simulink library "Multibody_Multiphysics_Lib"  (R2025a)
settings: Solver=ode45  StartTime=0.0  StopTime=10.0  RelTol=1e-3  EnableMultiTasking=on
undefined symbols (not defined in the file or in its folder): pst_rOut, rod_rOut
libraries: fl_lib x36, sm_lib x12, forcesPS_lib x9, $bdroot x1
Description:
  | Simscape Multibody Multiphysics Library v4.1
  | Copyright 2013-2025 The MathWorks, Inc.
settings Model: Creator=smiller  LastModifiedBy=smiller
settings SolverCC: AlgebraicLoopSolver=TrustRegion
settings DataIOCC: LimitDataPoints=on  SaveFormat=Array  SignalLoggingSaveFormat=ModelDataLogs  ReturnWorkspaceOutputs=off
settings OptimizationCC: ReuseModelBlockBuffer=off  ExpressionDepthLimit=2147483647.0  LifeSpan=inf
settings DebuggingCC: UnderspecifiedInitializationDetection=Classic  MergeDetectMultiDrivingBlocksExec=none  SolverPrmCheckMsg=warning  FcnCallInpInsideContextMsg=warning  UnconnectedInputMsg=warning  UnconnectedOutputMsg=warning  UnconnectedLineMsg=warning  AllowSymbolicDim=off  StateNameClashWarn=warning  PregeneratedLibrarySubsystemCodeDiagnostic=none  SFUnexpectedBacktrackingDiag=warning  SFNoUnconditionalDefaultTransitionDiag=warning  SFExecutionAtInitializationDiag=none  ArithmeticOperatorsInVariantConditions=warning
settings HardwareCC: ProdBitPerPointer=32.0  ProdBitPerSizeT=32.0  ProdBitPerPtrDiffT=32.0  ProdLargestAtomicFloat=None  ProdIntDivRoundTo=Undefined  ProdEndianess=Unspecified  ProdWordSize=32.0  ProdHWDeviceType=32-bit Generic
settings ModelReferenceCC: EnableRefExpFcnMdlSchedulingChecks=on  PropagateSignalLabelsOutOfModel=off
settings SFSimCC: SimUseLocalCustomCode=off  CustomCodeUndefinedFunction=UseInterfaceOnly
settings RTWCC: RTWUseLocalCustomCode=off  GPUComputeCapability=3.5  DLArmComputeVersion=19.05
settings CodeAppCC: StateflowObjectComments=on
settings GRTTargetCC: TargetLangStandard=C89/C90 (ANSI)
settings ConfigComp: CovMetricSettings=dw  CovSaveCumulativeToWorkspaceVar=on  CovSaveSingleToWorkspaceVar=on  CovExternalEMLEnable=off  CovSFcnEnable=off

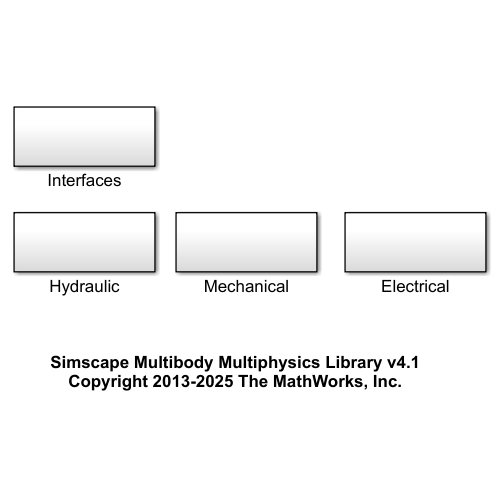
[thumbnail: Simulink's stored preview of the top-level diagram]
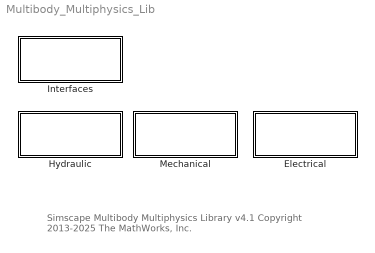
== system Multibody_Multiphysics_Lib ==
  note: Simscape Multibody Multiphysics Library v4.1
      | Copyright 2013-2025 The MathWorks, Inc.
  Electrical : Subsystem
  Hydraulic : Subsystem
  Interfaces : Subsystem
  Mechanical : Subsystem

== system Multibody_Multiphysics_Lib/Electrical ==
  DC Motor : Subsystem  Tag=PublishSubsystem

== system Multibody_Multiphysics_Lib/Hydraulic ==
  Hydraulic Actuator : Subsystem  mask(Double-Acting Hydraulic Cylinder, Kinematic Inputs){area_A=3e-4, area_B=1.57e-4, hs_stroke=0.1, hs_init_pos=0.01, dead_vol_A=1e-4, dead_vol_B=1e-4, popup_chamber_volume=Fixed, hs_stiffness=1e9, hs_damping=1500, friction_brkwy_frc=25, friction_brkwy_vel=0.1, friction_col_frc=20, friction_visc_coef=100}
      mask prompts: area_A "Piston Area A (m^2)"; area_B "Piston Area B (m^2)"; hs_stroke "Cylinder Stroke (m)"; hs_init_pos "Initial Position (m)"; dead_vol_A "Dead Volume Side A (m^3)"; dead_vol_B "Dead Volume Side B (m^3)"; popup_chamber_volume "Chamber Volume"; hs_stiffness "Hardstop Stiffness (N/m)"; hs_damping "Hardstop Damping (N/(m*s))"; friction_brkwy_frc "Breakaway Friction Force (N)"; friction_brkwy_vel "Breakaway Friction Velocity (m/s)"; friction_col_frc "Coulomb Friction Force (N)"; friction_visc_coef "Viscous Friction Coeff. (N/(m/s))"
      mask help:
      | Models a double-acting hydraulic cylinder with hardstops and compressibility.
      |
      | The position (m) and velocity (m/s) of the piston are inputs to this model.  This is to simplify the integration of this component with a Simscape Multibody joint.
      mask init:
      | temp_blk_h = gcb;
      | set_param([temp_blk_h '/Chamber A'],'dynamic_compressibility',num2str(popup_chamber_volume-1));
      | set_param([temp_blk_h '/Chamber B'],'dynamic_compressibility',num2str(popup_chamber_volume-1));
      | clear temp_blk_h
      mask TypeOptions popup_chamber_volume: Fixed | Varying
      mask DialogControl Container6 Prompt: Hydraulic
      mask DialogControl Container7 Prompt: Hardstop
      mask DialogControl Container8 Prompt: Friction
      mask Display:
      | color('white')
      | plot(-30,113.854429218918+10);
      | plot(326.445687096566+30,0);
      | color('black')
      | plot([127.790967235342;156.136468285695;156.136468285695;127.790967235342;127.790967235342], [113.618216710165;113.618216710165;56.927214609459;56.927214609459;113.618216710165])
      | plot([227.000220911577;227.000220911577;56.927214609459;56.927214609459;227.000220911577;227.000220911577], [99.4454661849886;113.618216710165;113.618216710165;56.927214609459;56.927214609459;71.0999651346356])
      | plot([156.136468285695;297.86397353746;297.86397353746;156.136468285695;156.136468285695], [99.4454661849886;99.4454661849886;71.0999651346356;71.0999651346356;99.4454661849886])
      | plot([56.927214609459;28.581713559106;56.927214609459], [113.618216710165;85.2727156598121;56.927214609459])
      | plot([28.581713559106;0.236212508752942], [85.2727156598121;85.2727156598121])
      | plot([297.86397353746;326.209474587813], [85.2727156598121;85.2727156598121])
      | plot([0.236212508752942;71.0999651346356;71.0999651346356], [28.581713559106;28.581713559106;56.927214609459])
      | plot([212.827470386401;212.827470386401;323.374924482778], [56.927214609459;28.581713559106;28.581713559106])
  Hydraulic Actuator PS FLib : Subsystem  Tag=PublishSubsystem  mask(Double-Acting Hydraulic Cylinder, PS Ports){area_A=pi*(pst_rOut/100)^2, area_B=pi*((pst_rOut/100)^2-(rod_rOut/100^2)), dead_vol_A=1e-4, dead_vol_B=1e-4, popup_chamber_volume=Fixed, p0_A=0, p0_B=0, friction_brkwy_frc=25, friction_brkwy_vel=0.1, friction_col_frc=20, friction_visc_coef=100}
      mask prompts: area_A "Piston Area A (m^2)"; area_B "Piston Area B (m^2)"; dead_vol_A "Dead Volume Side A (m^3)"; dead_vol_B "Dead Volume Side B (m^3)"; popup_chamber_volume "Chamber Volume"; p0_A "Initial Pressure A (Pa)"; p0_B "Initial Pressure B (Pa)"; friction_brkwy_frc "Breakaway Friction Force (N)"; friction_brkwy_vel "Breakaway Friction Velocity (m/s)"; friction_col_frc "Coulomb Friction Force (N)"; friction_visc_coef "Viscous Friction Coeff. (N/(m/s))"
      mask help:
      | Models a double-acting hydraulic cylinder with compressibility.
      |
      | The position (m) and velocity (m/s) of the piston are inputs to this model.  This is to simplify the integration of this component with a Simscape Multibody joint.
      mask init:
      | temp_blk_h = gcb;
      | set_param([temp_blk_h '/Chamber A'],'dynamic_compressibility',num2str(popup_chamber_volume-1));
      | set_param([temp_blk_h '/Chamber B'],'dynamic_compressibility',num2str(popup_chamber_volume-1));
      | clear temp_blk_h
      | 
      | % Parameter callback section
      mask TypeOptions popup_chamber_volume: Fixed | Varying
      mask DialogControl Container6 Prompt: Hydraulic
      mask DialogControl Container11 Prompt: Friction
      mask Display:
      | color('white')
      | plot(-30,113.854429218918+10);
      | plot(326.445687096566+30,0);
      | color('black')
      | plot([127.790967235342;156.136468285695;156.136468285695;127.790967235342;127.790967235342], [113.618216710165;113.618216710165;56.927214609459;56.927214609459;113.618216710165])
      | plot([227.000220911577;227.000220911577;56.927214609459;56.927214609459;227.000220911577;227.000220911577], [99.4454661849886;113.618216710165;113.618216710165;56.927214609459;56.927214609459;71.0999651346356])
      | plot([156.136468285695;297.86397353746;297.86397353746;156.136468285695;156.136468285695], [99.4454661849886;99.4454661849886;71.0999651346356;71.0999651346356;99.4454661849886])
      | plot([56.927214609459;28.581713559106;56.927214609459], [113.618216710165;85.2727156598121;56.927214609459])
      | plot([28.581713559106;0.236212508752942], [85.2727156598121;85.2727156598121])
      | plot([297.86397353746;326.209474587813], [85.2727156598121;85.2727156598121])
      | plot([0.236212508752942;71.0999651346356;71.0999651346356], [28.581713559106;28.581713559106;56.927214609459])
      | plot([212.827470386401;212.827470386401;323.374924482778], [56.927214609459;28.581713559106;28.581713559106])
  Hydraulic Actuator SA PS FLib : Subsystem  Tag=PublishSubsystem  mask(Double-Acting Hydraulic Cylinder, PS Ports){area_A=pi*(pst_rOut/100)^2, dead_vol_A=1e-4, popup_chamber_volume=Fixed, p0_A=0, friction_brkwy_frc=25, friction_brkwy_vel=0.1, friction_col_frc=20, friction_visc_coef=100}
      mask prompts: area_A "Piston Area A (m^2)"; dead_vol_A "Dead Volume Side A (m^3)"; popup_chamber_volume "Chamber Volume"; p0_A "Initial Pressure A (Pa)"; friction_brkwy_frc "Breakaway Friction Force (N)"; friction_brkwy_vel "Breakaway Friction Velocity (m/s)"; friction_col_frc "Coulomb Friction Force (N)"; friction_visc_coef "Viscous Friction Coeff. (N/(m/s))"
      mask help:
      | Models a double-acting hydraulic cylinder with hardstops and compressibility.
      |
      | The position (m) and velocity (m/s) of the piston are inputs to this model.  This is to simplify the integration of this component with a Simscape Multibody joint.
      mask init:
      | temp_blk_h = gcb;
      | set_param([temp_blk_h '/Chamber A'],'dynamic_compressibility',num2str(popup_chamber_volume-1));
      | clear temp_blk_h
      mask TypeOptions popup_chamber_volume: Fixed | Varying
      mask DialogControl Container6 Prompt: Hydraulic
      mask DialogControl Container11 Prompt: Friction
      mask Display:
      | color('white')
      | plot(-30,113.854429218918+10);
      | plot(326.445687096566+30,0);
      | color('black')
      | plot([127.790967235342;156.136468285695;156.136468285695;127.790967235342;127.790967235342], [113.618216710165;113.618216710165;56.927214609459;56.927214609459;113.618216710165])
      | plot([227.000220911577;227.000220911577;56.927214609459;56.927214609459;227.000220911577;227.000220911577], [99.4454661849886;113.618216710165;113.618216710165;56.927214609459;56.927214609459;71.0999651346356])
      | plot([156.136468285695;297.86397353746;297.86397353746;156.136468285695;156.136468285695], [99.4454661849886;99.4454661849886;71.0999651346356;71.0999651346356;99.4454661849886])
      | plot([56.927214609459;28.581713559106;56.927214609459], [113.618216710165;85.2727156598121;56.927214609459])
      | plot([28.581713559106;0.236212508752942], [85.2727156598121;85.2727156598121])
      | plot([297.86397353746;326.209474587813], [85.2727156598121;85.2727156598121])
      | plot([0.236212508752942;71.0999651346356;71.0999651346356], [28.581713559106;28.581713559106;56.927214609459])
      | plot([212.827470386401;212.827470386401;323.374924482778], [56.927214609459;28.581713559106;28.581713559106])

== system Multibody_Multiphysics_Lib/Interfaces ==
  Rotational Simscape Intf : Subsystem
  Rotational Simscape Multibody : Subsystem
  Translational Simscape Intf : Subsystem
  Translational Simscape Multibody : Subsystem

== system Multibody_Multiphysics_Lib/Mechanical ==
  Rotational Hard Stop Friction : Subsystem  Tag=PublishSubsystem  mask(Rotational Hard Stop and Friction, Multibody Ports){hs_upper_bnd=45*pi/180, hs_lower_bnd=-45*pi/180, hs_stiffness=1e6, hs_damping=1e2, friction_brkwy_trq=2.5, friction_brkwy_vel=0.1, friction_col_trq=2, friction_visc_coeff=0.001}
      mask prompts: hs_upper_bnd "Max Angular Position (rad)"; hs_lower_bnd "Min Angular Position (rad)"; hs_stiffness "Hardstop Stiffness (N*m/rad)"; hs_damping "Hardstop Damping (N*m/(rad/s))"; friction_brkwy_trq "Breakaway Friction Torque (N*m)"; friction_brkwy_vel "Breakaway Friction Velocity (rad/s)"; friction_col_trq "Coulomb Friction Torque (N*m)"; friction_visc_coeff "Viscous Friction Coeff. (N*m/(rad/s))"
      mask help:
      | Hardstops and friction for use with rotational degrees of freedom in Simscape Multibody.
      |
      | Connect the mechanical ports in parallel with a Simscape Multibody joint that has a rotational degree of freedom.
      |
      | 1. Connect B and F ports to joint B and F ports, respectively
      | 2. Orient joint frames so rotation range is (lower -- upper)
      mask DialogControl Container15 Prompt: Hardstop
      mask DialogControl Container16 Prompt: Friction
  Rotational Hard Stop Friction PS : Subsystem  Tag=PublishSubsystem  mask(Rotational Hard Stop and Friction, PS Ports){hs_upper_bnd=45*pi/180, hs_lower_bnd=-45*pi/180, hs_stiffness=1e6, hs_damping=1e2, friction_brkwy_trq=2.5, friction_brkwy_vel=0.1, friction_col_trq=2, friction_visc_coef=0.001}
      mask prompts: hs_upper_bnd "Max Angular Position (rad)"; hs_lower_bnd "Min Angular Position (rad)"; hs_stiffness "Hardstop Stiffness (N*m/rad)"; hs_damping "Hardstop Damping (N*m/(rad/s))"; friction_brkwy_trq "Breakaway Friction Torque (N*m)"; friction_brkwy_vel "Breakaway Friction Velocity (rad/s)"; friction_col_trq "Coulomb Friction Force (N*m)"; friction_visc_coef "Viscous Friction Coeff. (N*m/(rad/s))"
      mask help:
      | Hardstops and friction force for use with rotational degrees of freedom in Simscape Multibody.
      |
      | Connect the physical signal ports to measurements from a Simscape Multibody joint with a rotational degree of freedom.  Apply the calculated torque to the frames used in the joint, either via joint actuation or torque blocks.
      |
      | 1. Connect B and F ports to joint B and F ports, respectively
      | 2. Orient joint frames so extension range is (0 -- stroke)
      mask DialogControl Container15 Prompt: Hardstop
      mask DialogControl Container16 Prompt: Friction
  Translational Hard Stop Friction : Subsystem  Tag=PublishSubsystem  mask(Translational Hard Stop and Friction, Multibody Ports){stroke=0.7, stiffness=1e9, damping=1.5e8, friction_breakaway=0.2, friction_brkwy_vel=0.1, friction_coulomb=0.2, friction_viscous=1*0.01}
      mask prompts: stroke "Distance Between Stops (m)"; stiffness "Hardstop Stiffness (N/m)"; damping "Hardstop Damping (N/(m*s))"; friction_breakaway "Breakaway Friction Force (N)"; friction_brkwy_vel "Breakaway Friction Velocity (m/s)"; friction_coulomb "Coulomb Friction Force (N)"; friction_viscous "Viscous Friction Coeff. (N/(m/s))"
      mask help:
      | Hardstops and friction for use with translational degrees of freedom in Simscape Multibody.
      |
      | Connect the mechanical ports in parallel with a Simscape Multibody joint that has a translational degree of freedom.
      |
      | 1. Connect B and F ports to joint B and F ports, respectively
      | 2. Orient joint frames so extension range is (0 -- distance)
      mask DialogControl Container15 Prompt: Hardstop
      mask DialogControl Container16 Prompt: Friction
  Translational Hard Stop Friction PS : Subsystem  mask(Translational Hard Stop and Friction, PS Ports){hs_stroke=0.1, hs_stiffness=1e6, hs_damping=1500, friction_brkwy_frc=25, friction_brkwy_vel=0.1, friction_col_frc=20, friction_visc_coef=100}
      mask prompts: hs_stroke "Distance between stops (m)"; hs_stiffness "Hardstop Stiffness (N/m)"; hs_damping "Hardstop Damping (N/(m*s))"; friction_brkwy_frc "Breakaway Friction Force (N)"; friction_brkwy_vel "Breakaway Friction Velocity (m/s)"; friction_col_frc "Coulomb Friction Force (N)"; friction_visc_coef "Viscous Friction Coeff. (N/(m/s))"
      mask help:
      | Hardstops and friction force for use with translational degrees of freedom in Simscape Multibody.
      |
      | Connect the physical signal ports to measurements from a Simscape Multibody joint with a translational degree of freedom.  Apply the calculated force to the frames used in the joint, either via joint actuation or force blocks.
      |
      | 1. Connect B and F ports to joint B and F ports, respectively
      | 2. Orient joint frames so extension range is (0 -- distance)
      mask DialogControl Container15 Prompt: Hardstop
      mask DialogControl Container16 Prompt: Friction

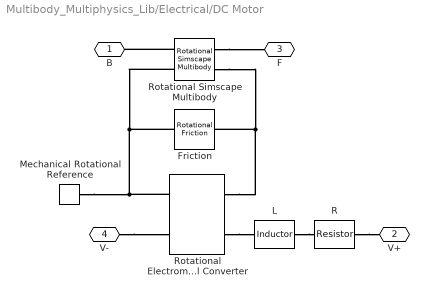
== system Multibody_Multiphysics_Lib/Electrical/DC Motor ==
  Friction : fl_lib/Mechanical/Rotational Elements/Rotational Friction  brkwy_trq=15e-3 N*m  brkwy_vel=0.057625 rad/s  Col_trq=5e-3 N*m  visc_coef=5e-3 N*m/(rad/s)  w_specify=off  w_priority=High  w=0 rad/s  w_nominal_specify=off  w_nominal_value=1  w_nominal_unit=rad/s  t_specify=off  t_priority=High  t=0 N*m  t_nominal_specify=off  t_nominal_value=1  t_nominal_unit=N*m
  L : fl_lib/Electrical/Electrical Elements/Inductor  l=12e-6 H  r=0 Ohm  g=1e-09 1/Ohm  i_specify=off  i_priority=High  i=0 A  i_nominal_specify=off  i_nominal_value=1  i_nominal_unit=A  v_specify=off  v_priority=High  v=0 V  v_nominal_specify=off  v_nominal_value=1  v_nominal_unit=V  i_L_specify=on  i_L_priority=High  i_L=0 A  i_L_nominal_specify=off  i_L_nominal_value=1  i_L_nominal_unit=A
  Mechanical Rotational Reference : fl_lib/Mechanical/Rotational Elements/Mechanical Rotational Reference
  R : fl_lib/Electrical/Electrical Elements/Resistor  Tag=Factory Generic  R=3.9 Ohm  i_specify=off  i_priority=High  i=0 A  i_nominal_specify=off  i_nominal_value=1  i_nominal_unit=A  v_specify=off  v_priority=High  v=0 V  v_nominal_specify=off  v_nominal_value=1  v_nominal_unit=V
  Rotational Electromechanical Converter : fl_lib/Electrical/Electrical Elements/Rotational Electromechanical Converter  K=0.072e-3*60/(2*pi)*20 V/(rad/s)  i_specify=off  i_priority=High  i=0 A  i_nominal_specify=off  i_nominal_value=1  i_nominal_unit=A  v_specify=off  v_priority=High  v=0 V  v_nominal_specify=off  v_nominal_value=1  v_nominal_unit=V  t_specify=off  t_priority=High  t=0 N*m  t_nominal_specify=off  t_nominal_value=1  t_nominal_unit=N*m  w_specify=off  w_priority=High  w=0 rad/s  w_nominal_specify=off  w_nominal_value=1  w_nominal_unit=rad/s
  Rotational Simscape Multibody : $bdroot/Interfaces/Rotational Simscape Multibody  Tag=PublishSubsystem  SystemSampleTime=-1  VariantActivationTime=update diagram  EmptyChoice=off  PassThrough=off  PassThroughVariantControl=(default)  EmptyChoiceVariantControl=(default)  AllowFlexibleInterface=on  Latency=0  AutoFrameSizeCalculation=off
  B : PMIOPort  Side=Left
  V+ : PMIOPort  Port=2  Side=Left
  F : PMIOPort  Port=3  Side=Right
  V- : PMIOPort  Port=4  Side=Right
  connections:
  Rotational Simscape Multibody/LConn1 -- B/RConn1
  Rotational Simscape Multibody/RConn1 -- F/RConn1
  Rotational Electromechanical Converter/LConn1 -- L/RConn1
  V-/RConn1 -- Rotational Electromechanical Converter/RConn1
  R/LConn1 -- V+/RConn1
  L/LConn1 -- R/RConn1
  Rotational Electromechanical Converter/LConn2 -- Rotational Simscape Multibody/RConn2 -- Friction/LConn1
  Mechanical Rotational Reference/LConn1 -- Rotational Electromechanical Converter/RConn2 -- Rotational Simscape Multibody/LConn2 -- Friction/RConn1

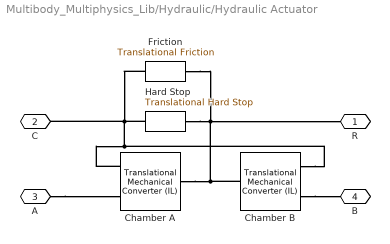
== system Multibody_Multiphysics_Lib/Hydraulic/Hydraulic Actuator ==
  Chamber A : fl_lib/Isothermal Liquid/Elements/Translational Mechanical Converter (IL)  mech_orientation=1  displacement_spec=foundation.enum.DisplacementSpec.Calculate  x0=hs_init_pos m  interface_area=area_A m^2  dead_volume=dead_vol_A m^3  pressure_spec=1  environment_pressure=0.101325 MPa  dynamic_compressibility=0  p0=0 + 101325 Pa  p_nominal=0.101325 MPa
      settings: InternalSimscapePortConfiguration="{\"Bottom\":[],\"Left\":[{\"id\":\"A\",\"label\":\"A\",\"type\":\"foundation.isothermal_liquid.isothermal_liquid\"},{\"id\":\"C\",\"label\":\"C\",\"type\":\"foundation.mechanical.translational.translational\"}],\"Right\":[{\"id\":\"R\",\"label\":\"R\",\"type\":\"foundation.mechanical.translational.translational\"}],\"Top\":[]}"
      settings: LibrarySourceBlock=|
      | fl_lib/Hydraulic/Hydraulic Elements/Translational
      | Hydro-Mechanical
      | Converter
  Chamber B : fl_lib/Isothermal Liquid/Elements/Translational Mechanical Converter (IL)  mech_orientation=-1  displacement_spec=foundation.enum.DisplacementSpec.Calculate  x0=-(hs_stroke - hs_init_pos) m  interface_area=area_B m^2  dead_volume=dead_vol_B m^3  pressure_spec=1  environment_pressure=0.101325 MPa  dynamic_compressibility=0  p0=0 + 101325 Pa  p_nominal=0.101325 MPa
      settings: InternalSimscapePortConfiguration="{\"Bottom\":[],\"Left\":[{\"id\":\"A\",\"label\":\"A\",\"type\":\"foundation.isothermal_liquid.isothermal_liquid\"},{\"id\":\"C\",\"label\":\"C\",\"type\":\"foundation.mechanical.translational.translational\"}],\"Right\":[{\"id\":\"R\",\"label\":\"R\",\"type\":\"foundation.mechanical.translational.translational\"}],\"Top\":[]}"
      settings: LibrarySourceBlock=|
      | fl_lib/Hydraulic/Hydraulic Elements/Translational
      | Hydro-Mechanical
      | Converter
  Friction : fl_lib/Mechanical/Translational Elements/Translational Friction  brkwy_frc=friction_brkwy_frc N  brkwy_vel=friction_brkwy_vel m/s  Col_frc=friction_col_frc N  visc_coef=friction_visc_coef N/(m/s)  v_specify=off  v_priority=None  v=0 m/s  v_nominal_specify=off  v_nominal_value=1  v_nominal_unit=m/s  f_specify=off  f_priority=None  f=0 N  f_nominal_specify=off  f_nominal_value=1  f_nominal_unit=N
      settings: InternalSimscapePortConfiguration="{\"Bottom\":[],\"Left\":[{\"id\":\"R\",\"label\":\"R\",\"type\":\"foundation.mechanical.translational.translational\"}],\"Right\":[{\"id\":\"C\",\"label\":\"C\",\"type\":\"foundation.mechanical.translational.translational\"}],\"Top\":[]}"
  Hard Stop : fl_lib/Mechanical/Translational Elements/Translational Hard Stop  upper_bnd=hs_stroke - hs_init_pos m  lower_bnd=-hs_init_pos m  model=3  stiff_up=hs_stiffness N/m  stiff_low=hs_stiffness N/m  D_up=hs_damping N/(m/s)  D_low=hs_damping N/(m/s)  transition=0.1 mm  coeff_rest=0.7  v_tol=0.001 m/s  f_tol=0.001 N  v_specify=off  v_priority=High  v=0 m/s  v_nominal_specify=off  v_nominal_value=1  v_nominal_unit=m/s  f_specify=off  f_priority=High  f=0 N  f_nominal_specify=off  f_nominal_value=1  f_nominal_unit=N  x_specify=on  x_priority=High  x=0 m  x_nominal_specify=off  x_nominal_value=1  x_nominal_unit=m  M_specify=off  M_priority=None  M=0
  R : PMIOPort  Tag=CustomStyle  Side=Right
  C : PMIOPort  Tag=CustomStyle  Port=2  Side=Left
  A : PMIOPort  Tag=PMCPort  Port=3  Side=Left
  B : PMIOPort  Tag=PMCPort  Port=4  Side=Right
  connections:
  A/RConn1 -- Chamber A/LConn1
  Friction/RConn1 -- Chamber B/LConn2 -- Chamber A/LConn2 -- C/RConn1 -- Hard Stop/RConn1
  Hard Stop/LConn1 -- R/RConn1 -- Friction/LConn1 -- Chamber B/RConn1 -- Chamber A/RConn1
  Chamber B/LConn1 -- B/RConn1

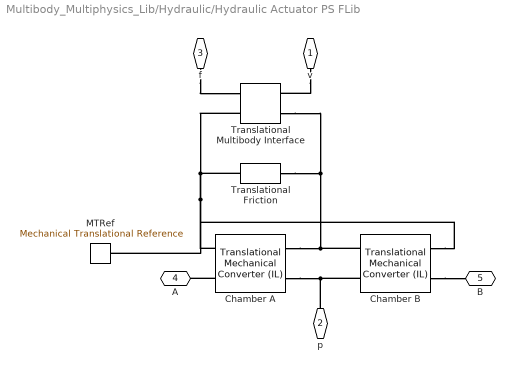
== system Multibody_Multiphysics_Lib/Hydraulic/Hydraulic Actuator PS FLib ==
  Chamber A : fl_lib/Isothermal Liquid/Elements/Translational Mechanical Converter (IL)  mech_orientation=1  displacement_spec=foundation.enum.DisplacementSpec.InputSignal  x0=0 m  interface_area=area_A m^2  dead_volume=dead_vol_A m^3  pressure_spec=1  environment_pressure=0.101325 MPa  dynamic_compressibility=0  p0=p0_A + 101325 Pa  p_nominal=0.101325 MPa
      settings: InternalSimscapePortConfiguration="{\"Bottom\":[],\"Left\":[{\"id\":\"A\",\"label\":\"A\",\"type\":\"foundation.isothermal_liquid.isothermal_liquid\"},{\"id\":\"C\",\"label\":\"C\",\"type\":\"foundation.mechanical.translational.translational\"}],\"Right\":[{\"id\":\"p_in\",\"label\":\"p\",\"type\":\"input\"},{\"id\":\"R\",\"label\":\"R\",\"type\":\"foundation.mechanical.translational.translational\"}],\"Top\":[]}"
      settings: LibrarySourceBlock=|
      | fl_lib/Hydraulic/Hydraulic Elements/Translational
      | Hydro-Mechanical
      | Converter
  Chamber B : fl_lib/Isothermal Liquid/Elements/Translational Mechanical Converter (IL)  mech_orientation=-1  displacement_spec=foundation.enum.DisplacementSpec.InputSignal  x0=-(0) m  interface_area=area_B m^2  dead_volume=dead_vol_B m^3  pressure_spec=1  environment_pressure=0.101325 MPa  dynamic_compressibility=0  p0=p0_B + 101325 Pa  p_nominal=0.101325 MPa
      settings: InternalSimscapePortConfiguration="{\"Bottom\":[],\"Left\":[{\"id\":\"A\",\"label\":\"A\",\"type\":\"foundation.isothermal_liquid.isothermal_liquid\"},{\"id\":\"C\",\"label\":\"C\",\"type\":\"foundation.mechanical.translational.translational\"}],\"Right\":[{\"id\":\"p_in\",\"label\":\"p\",\"type\":\"input\"},{\"id\":\"R\",\"label\":\"R\",\"type\":\"foundation.mechanical.translational.translational\"}],\"Top\":[]}"
      settings: LibrarySourceBlock=|
      | fl_lib/Hydraulic/Hydraulic Elements/Translational
      | Hydro-Mechanical
      | Converter
  MTRef : fl_lib/Mechanical/Translational Elements/Mechanical Translational Reference
  Translational Friction : fl_lib/Mechanical/Translational Elements/Translational Friction  brkwy_frc=friction_brkwy_frc N  brkwy_vel=friction_brkwy_vel m/s  Col_frc=friction_col_frc N  visc_coef=friction_visc_coef N/(m/s)  v_specify=off  v_priority=None  v=0 m/s  v_nominal_specify=off  v_nominal_value=1  v_nominal_unit=m/s  f_specify=off  f_priority=None  f=0 N  f_nominal_specify=off  f_nominal_value=1  f_nominal_unit=N
      settings: InternalSimscapePortConfiguration="{\"Bottom\":[],\"Left\":[{\"id\":\"R\",\"label\":\"R\",\"type\":\"foundation.mechanical.translational.translational\"}],\"Right\":[{\"id\":\"C\",\"label\":\"C\",\"type\":\"foundation.mechanical.translational.translational\"}],\"Top\":[]}"
  Translational Multibody Interface : fl_lib/Mechanical/Multibody Interfaces/Translational Multibody Interface
  v : PMIOPort  Side=Right
  p : PMIOPort  Port=2  Side=Right
  f : PMIOPort  Port=3  Side=Left
  A : PMIOPort  Port=4  Side=Left
  B : PMIOPort  Port=5  Side=Right
  connections:
  f/RConn1 -- Translational Multibody Interface/LConn1
  v/RConn1 -- Translational Multibody Interface/RConn1
  Translational Friction/LConn1 -- Chamber B/RConn2 -- Chamber A/RConn2 -- Translational Multibody Interface/RConn2
  Chamber A/LConn1 -- A/RConn1
  Translational Friction/RConn1 -- Chamber B/LConn2 -- MTRef/LConn1 -- Chamber A/LConn2 -- Translational Multibody Interface/LConn2
  p/RConn1 -- Chamber B/RConn1 -- Chamber A/RConn1
  Chamber B/LConn1 -- B/RConn1

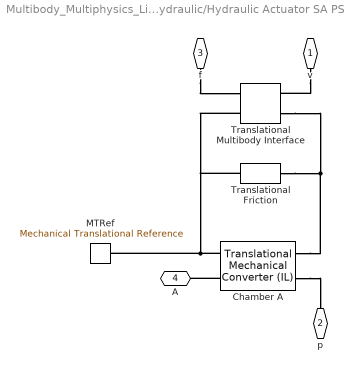
== system Multibody_Multiphysics_Lib/Hydraulic/Hydraulic Actuator SA PS FLib ==
  Chamber A : fl_lib/Isothermal Liquid/Elements/Translational Mechanical Converter (IL)  mech_orientation=1  displacement_spec=foundation.enum.DisplacementSpec.InputSignal  x0=0 m  interface_area=area_A m^2  dead_volume=dead_vol_A m^3  pressure_spec=1  environment_pressure=0.101325 MPa  dynamic_compressibility=0  p0=p0_A + 101325 Pa  p_nominal=0.101325 MPa
      settings: InternalSimscapePortConfiguration="{\"Bottom\":[],\"Left\":[{\"id\":\"A\",\"label\":\"A\",\"type\":\"foundation.isothermal_liquid.isothermal_liquid\"},{\"id\":\"C\",\"label\":\"C\",\"type\":\"foundation.mechanical.translational.translational\"}],\"Right\":[{\"id\":\"p_in\",\"label\":\"p\",\"type\":\"input\"},{\"id\":\"R\",\"label\":\"R\",\"type\":\"foundation.mechanical.translational.translational\"}],\"Top\":[]}"
      settings: LibrarySourceBlock=|
      | fl_lib/Hydraulic/Hydraulic Elements/Translational
      | Hydro-Mechanical
      | Converter
  MTRef : fl_lib/Mechanical/Translational Elements/Mechanical Translational Reference
  Translational Friction : fl_lib/Mechanical/Translational Elements/Translational Friction  brkwy_frc=friction_brkwy_frc N  brkwy_vel=friction_brkwy_vel m/s  Col_frc=friction_col_frc N  visc_coef=friction_visc_coef N/(m/s)  v_specify=off  v_priority=None  v=0 m/s  v_nominal_specify=off  v_nominal_value=1  v_nominal_unit=m/s  f_specify=off  f_priority=None  f=0 N  f_nominal_specify=off  f_nominal_value=1  f_nominal_unit=N
      settings: InternalSimscapePortConfiguration="{\"Bottom\":[],\"Left\":[{\"id\":\"R\",\"label\":\"R\",\"type\":\"foundation.mechanical.translational.translational\"}],\"Right\":[{\"id\":\"C\",\"label\":\"C\",\"type\":\"foundation.mechanical.translational.translational\"}],\"Top\":[]}"
  Translational Multibody Interface : fl_lib/Mechanical/Multibody Interfaces/Translational Multibody Interface
  v : PMIOPort  Side=Right
  p : PMIOPort  Port=2  Side=Right
  f : PMIOPort  Port=3  Side=Left
  A : PMIOPort  Port=4  Side=Left
  connections:
  v/RConn1 -- Translational Multibody Interface/RConn1
  f/RConn1 -- Translational Multibody Interface/LConn1
  Translational Multibody Interface/LConn2 -- Translational Friction/RConn1 -- Chamber A/LConn2 -- MTRef/LConn1
  Translational Friction/LConn1 -- Chamber A/RConn2 -- Translational Multibody Interface/RConn2
  Chamber A/LConn1 -- A/RConn1
  Chamber A/RConn1 -- p/RConn1

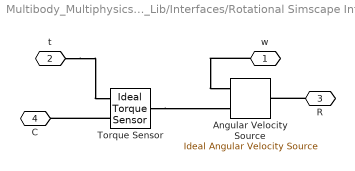
== system Multibody_Multiphysics_Lib/Interfaces/Rotational Simscape Intf ==
  Angular Velocity Source : fl_lib/Mechanical/Mechanical Sources/Ideal Angular Velocity Source
  Torque Sensor : fl_lib/Mechanical/Mechanical Sensors/Ideal Torque Sensor
  w : PMIOPort  Side=Right
  t : PMIOPort  Port=2  Side=Left
  R : PMIOPort  Port=3  Side=Right
  C : PMIOPort  Port=4  Side=Left
  connections:
  w/RConn1 -- Angular Velocity Source/RConn1
  t/RConn1 -- Torque Sensor/RConn2
  Torque Sensor/LConn1 -- Angular Velocity Source/RConn2
  R/RConn1 -- Angular Velocity Source/LConn1
  Torque Sensor/RConn1 -- C/RConn1

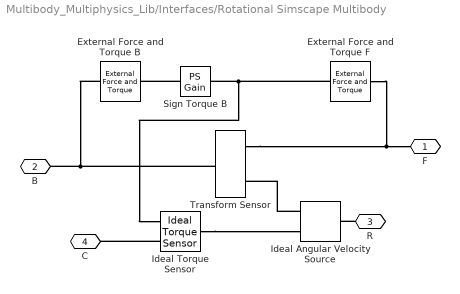
== system Multibody_Multiphysics_Lib/Interfaces/Rotational Simscape Multibody ==
  External Force and Torque B : sm_lib/Forces and Torques/External Force and Torque  EnableForceX=off  EnableForceY=off  EnableForceZ=off  EnableForce=off  ForceResolutionFrame=AttachedFrame  EnableTorqueX=off  EnableTorqueY=off  EnableTorqueZ=on  EnableTorque=off  TorqueResolutionFrame=AttachedFrame
  External Force and Torque F : sm_lib/Forces and Torques/External Force and Torque  EnableForceX=off  EnableForceY=off  EnableForceZ=off  EnableForce=off  ForceResolutionFrame=AttachedFrame  EnableTorqueX=off  EnableTorqueY=off  EnableTorqueZ=on  EnableTorque=off  TorqueResolutionFrame=AttachedFrame
  Ideal Angular Velocity Source : fl_lib/Mechanical/Mechanical Sources/Ideal Angular Velocity Source
  Ideal Torque Sensor : fl_lib/Mechanical/Mechanical Sensors/Ideal Torque Sensor
  Sign Torque B : fl_lib/Physical Signals/Functions/PS Gain  gain=-1
  Transform Sensor : sm_lib/Frames and Transforms/Transform Sensor  MeasurementFrame=Base  RotationSequence=XYX  SenseAngle=off  SenseAxis=off  SenseQ=off  SenseR=off  SenseRotationSequence=off  SenseOmegaX=off  SenseOmegaY=off  SenseOmegaZ=on  SenseOmega=off  SenseQDot=off  SenseRDot=off  SenseRotationSequenceDot=off  SenseAlphaX=off  SenseAlphaY=off  SenseAlphaZ=off  SenseAlpha=off  SenseQDDot=off  SenseRDDot=off  SenseX=off  SenseY=off  SenseZ=off  SenseXYZ=off  SenseRad=off  SenseAzim=off  SenseDist=off  SenseInc=off  SenseXDot=off  SenseYDot=off  SenseZDot=off  SenseXYZDot=off  SenseRadDot=off  SenseAzimDot=off  SenseDistDot=off  SenseIncDot=off  SenseXDDot=off  SenseYDDot=off  SenseZDDot=off  SenseXYZDDot=off  SenseRadDDot=off  SenseAzimDDot=off  SenseDistDDot=off  SenseIncDDot=off
  F : PMIOPort  Side=Right
  B : PMIOPort  Port=2  Side=Left
  R : PMIOPort  Port=3  Side=Right
  C : PMIOPort  Port=4  Side=Left
  connections:
  Ideal Torque Sensor/RConn1 -- C/RConn1
  R/RConn1 -- Ideal Angular Velocity Source/LConn1
  Ideal Torque Sensor/LConn1 -- Ideal Angular Velocity Source/RConn2
  Transform Sensor/LConn1 -- B/RConn1 -- External Force and Torque B/RConn1
  Transform Sensor/RConn1 -- External Force and Torque F/RConn1 -- F/RConn1
  Ideal Angular Velocity Source/RConn1 -- Transform Sensor/RConn2
  Sign Torque B/RConn1 -- External Force and Torque B/LConn1
  External Force and Torque F/LConn1 -- Ideal Torque Sensor/RConn2 -- Sign Torque B/LConn1

== system Multibody_Multiphysics_Lib/Interfaces/Translational Simscape Intf ==
  Force Sensor : fl_lib/Mechanical/Mechanical Sensors/Ideal Force Sensor
  Velocity Source : fl_lib/Mechanical/Mechanical Sources/Ideal Translational Velocity Source
  v : PMIOPort  Side=Right
  f : PMIOPort  Port=2  Side=Left
  R : PMIOPort  Port=3  Side=Right
  C : PMIOPort  Port=4  Side=Left
  connections:
  Force Sensor/RConn1 -- C/RConn1
  R/RConn1 -- Velocity Source/LConn1
  Force Sensor/LConn1 -- Velocity Source/RConn2
  f/RConn1 -- Force Sensor/RConn2
  v/RConn1 -- Velocity Source/RConn1

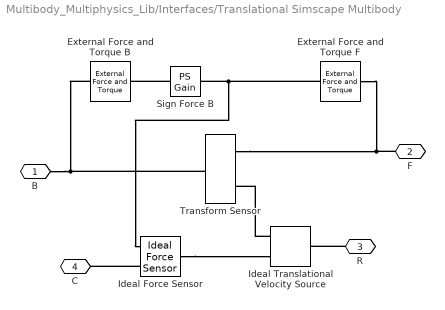
== system Multibody_Multiphysics_Lib/Interfaces/Translational Simscape Multibody ==
  External Force and Torque B : sm_lib/Forces and Torques/External Force and Torque  EnableForceX=off  EnableForceY=off  EnableForceZ=on  EnableForce=off  ForceResolutionFrame=AttachedFrame  EnableTorqueX=off  EnableTorqueY=off  EnableTorqueZ=off  EnableTorque=off  TorqueResolutionFrame=AttachedFrame
  External Force and Torque F : sm_lib/Forces and Torques/External Force and Torque  EnableForceX=off  EnableForceY=off  EnableForceZ=on  EnableForce=off  ForceResolutionFrame=AttachedFrame  EnableTorqueX=off  EnableTorqueY=off  EnableTorqueZ=off  EnableTorque=off  TorqueResolutionFrame=AttachedFrame
  Ideal Force Sensor : fl_lib/Mechanical/Mechanical Sensors/Ideal Force Sensor
  Ideal Translational Velocity Source : fl_lib/Mechanical/Mechanical Sources/Ideal Translational Velocity Source
  Sign Force B : fl_lib/Physical Signals/Functions/PS Gain  gain=-1
  Transform Sensor : sm_lib/Frames and Transforms/Transform Sensor  MeasurementFrame=Base  RotationSequence=XYX  SenseAngle=off  SenseAxis=off  SenseQ=off  SenseR=off  SenseRotationSequence=off  SenseOmegaX=off  SenseOmegaY=off  SenseOmegaZ=off  SenseOmega=off  SenseQDot=off  SenseRDot=off  SenseRotationSequenceDot=off  SenseAlphaX=off  SenseAlphaY=off  SenseAlphaZ=off  SenseAlpha=off  SenseQDDot=off  SenseRDDot=off  SenseX=off  SenseY=off  SenseZ=off  SenseXYZ=off  SenseRad=off  SenseAzim=off  SenseDist=off  SenseInc=off  SenseXDot=off  SenseYDot=off  SenseZDot=on  SenseXYZDot=off  SenseRadDot=off  SenseAzimDot=off  SenseDistDot=off  SenseIncDot=off  SenseXDDot=off  SenseYDDot=off  SenseZDDot=off  SenseXYZDDot=off  SenseRadDDot=off  SenseAzimDDot=off  SenseDistDDot=off  SenseIncDDot=off
  B : PMIOPort  Side=Left
  F : PMIOPort  Port=2  Side=Right
  R : PMIOPort  Port=3  Side=Right
  C : PMIOPort  Port=4  Side=Left
  connections:
  Ideal Translational Velocity Source/RConn1 -- Transform Sensor/RConn2
  Sign Force B/LConn1 -- Ideal Force Sensor/RConn2 -- External Force and Torque F/LConn1
  Ideal Force Sensor/LConn1 -- Ideal Translational Velocity Source/RConn2
  R/RConn1 -- Ideal Translational Velocity Source/LConn1
  Ideal Force Sensor/RConn1 -- C/RConn1
  External Force and Torque B/RConn1 -- B/RConn1 -- Transform Sensor/LConn1
  External Force and Torque F/RConn1 -- F/RConn1 -- Transform Sensor/RConn1
  Sign Force B/RConn1 -- External Force and Torque B/LConn1

== system Multibody_Multiphysics_Lib/Mechanical/Rotational Hard Stop Friction ==
  Friction : forcesPS_lib/Mechanical/Rotational Friction Force  brkwy_trq=friction_brkwy_trq N*m  brkwy_vel=friction_brkwy_vel rad/s  Col_trq=friction_col_trq N*m  visc_coef=friction_visc_coeff N*m/(rad/s)
      settings: InternalSimscapePortConfiguration="{\"Bottom\":[],\"Left\":[{\"id\":\"w\",\"label\":\"w\",\"type\":\"input\"}],\"Right\":[{\"id\":\"t\",\"label\":\"t\",\"type\":\"output\"}],\"Top\":[]}"
  Hard Stop : forcesPS_lib/Mechanical/Rotational Hard Stop Force  upper_bnd=hs_upper_bnd rad  lower_bnd=hs_lower_bnd rad  stiff_up=hs_stiffness N*m/rad  stiff_low=hs_stiffness N*m/rad  D_up=hs_damping N*m/(rad/s)  D_low=hs_damping N*m/(rad/s)
      settings: InternalSimscapePortConfiguration="{\"Bottom\":[],\"Left\":[{\"id\":\"w\",\"label\":\"w\",\"type\":\"input\"},{\"id\":\"phi\",\"label\":\"q\",\"type\":\"input\"}],\"Right\":[{\"id\":\"t\",\"label\":\"t\",\"type\":\"output\"}],\"Top\":[]}"
  Interface 3D-1D : Subsystem
  PS Add Friction : fl_lib/Physical Signals/Functions/PS Add
  B : PMIOPort  Tag=CustomStyle  Side=Left
  F : PMIOPort  Tag=CustomStyle  Port=2  Side=Right
  connections:
  Hard Stop/RConn1 -- PS Add Friction/LConn1
  Interface 3D-1D/LConn2 -- Hard Stop/LConn2
  Interface 3D-1D/RConn2 -- PS Add Friction/RConn1
  Interface 3D-1D/LConn1 -- B/RConn1
  Interface 3D-1D/RConn1 -- F/RConn1
  Friction/RConn1 -- PS Add Friction/LConn2
  Interface 3D-1D/LConn3 -- Hard Stop/LConn1 -- Friction/LConn1

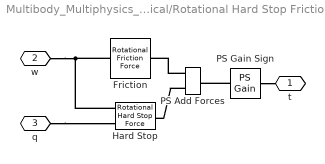
== system Multibody_Multiphysics_Lib/Mechanical/Rotational Hard Stop Friction PS ==
  Friction : forcesPS_lib/Mechanical/Rotational Friction Force  brkwy_trq=friction_brkwy_trq N*m  brkwy_vel=friction_brkwy_vel rad/s  Col_trq=friction_col_trq N*m  visc_coef=friction_visc_coef N*m/(rad/s)
      settings: InternalSimscapePortConfiguration="{\"Bottom\":[],\"Left\":[{\"id\":\"w\",\"label\":\"w\",\"type\":\"input\"}],\"Right\":[{\"id\":\"t\",\"label\":\"t\",\"type\":\"output\"}],\"Top\":[]}"
  Hard Stop : forcesPS_lib/Mechanical/Rotational Hard Stop Force  upper_bnd=hs_upper_bnd rad  lower_bnd=hs_lower_bnd rad  stiff_up=hs_stiffness N*m/rad  stiff_low=hs_stiffness N*m/rad  D_up=hs_damping N*m/(rad/s)  D_low=hs_damping N*m/(rad/s)
      settings: InternalSimscapePortConfiguration="{\"Bottom\":[],\"Left\":[{\"id\":\"w\",\"label\":\"w\",\"type\":\"input\"},{\"id\":\"phi\",\"label\":\"q\",\"type\":\"input\"}],\"Right\":[{\"id\":\"t\",\"label\":\"t\",\"type\":\"output\"}],\"Top\":[]}"
  PS Add Forces : fl_lib/Physical Signals/Functions/PS Add
  PS Gain Sign : fl_lib/Physical Signals/Functions/PS Gain  gain=-1
  t : PMIOPort  Side=Left
  w : PMIOPort  Port=2  Side=Right
  q : PMIOPort  Port=3  Side=Right
  connections:
  PS Add Forces/LConn2 -- Hard Stop/RConn1
  q/RConn1 -- Hard Stop/LConn2
  PS Add Forces/LConn1 -- Friction/RConn1
  Hard Stop/LConn1 -- Friction/LConn1 -- w/RConn1
  PS Gain Sign/RConn1 -- t/RConn1
  PS Gain Sign/LConn1 -- PS Add Forces/RConn1

== system Multibody_Multiphysics_Lib/Mechanical/Translational Hard Stop Friction ==
  Friction : forcesPS_lib/Mechanical/Translational Friction Force  brkwy_frc=friction_breakaway N  brkwy_vel=friction_brkwy_vel m/s  Col_frc=friction_coulomb N  visc_coef=friction_viscous N/(m/s)
      settings: InternalSimscapePortConfiguration="{\"Bottom\":[],\"Left\":[{\"id\":\"v\",\"label\":\"v\",\"type\":\"input\"}],\"Right\":[{\"id\":\"f\",\"label\":\"f\",\"type\":\"output\"}],\"Top\":[]}"
  Hard Stop : forcesPS_lib/Mechanical/Translational Hard Stop Force  upper_bnd=stroke m  lower_bnd=0 m  stiff_up=stiffness N/m  stiff_low=stiffness N/m  D_up=damping N/(m/s)  D_low=damping N/(m/s)
      settings: InternalSimscapePortConfiguration="{\"Bottom\":[],\"Left\":[{\"id\":\"v\",\"label\":\"v\",\"type\":\"input\"},{\"id\":\"p\",\"label\":\"p\",\"type\":\"input\"}],\"Right\":[{\"id\":\"f\",\"label\":\"f\",\"type\":\"output\"}],\"Top\":[]}"
  Interface 3D-1D : Subsystem
  PS Add Friction : fl_lib/Physical Signals/Functions/PS Add
  B : PMIOPort  Tag=CustomStyle  Side=Left
  F : PMIOPort  Tag=CustomStyle  Port=2  Side=Right
  connections:
  Hard Stop/LConn2 -- Interface 3D-1D/LConn2
  Friction/LConn1 -- Interface 3D-1D/LConn3 -- Hard Stop/LConn1
  Hard Stop/RConn1 -- PS Add Friction/LConn1
  Friction/RConn1 -- PS Add Friction/LConn2
  Interface 3D-1D/RConn1 -- F/RConn1
  Interface 3D-1D/LConn1 -- B/RConn1
  Interface 3D-1D/RConn2 -- PS Add Friction/RConn1

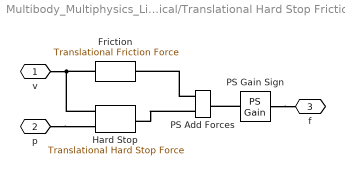
== system Multibody_Multiphysics_Lib/Mechanical/Translational Hard Stop Friction PS ==
  Friction : forcesPS_lib/Mechanical/Translational Friction Force  brkwy_frc=friction_brkwy_frc N  brkwy_vel=friction_brkwy_vel m/s  Col_frc=friction_col_frc N  visc_coef=friction_visc_coef N/(m/s)
      settings: InternalSimscapePortConfiguration="{\"Bottom\":[],\"Left\":[{\"id\":\"v\",\"label\":\"v\",\"type\":\"input\"}],\"Right\":[{\"id\":\"f\",\"label\":\"f\",\"type\":\"output\"}],\"Top\":[]}"
  Hard Stop : forcesPS_lib/Mechanical/Translational Hard Stop Force  upper_bnd=hs_stroke m  lower_bnd=0 m  stiff_up=hs_stiffness N/m  stiff_low=hs_stiffness N/m  D_up=hs_damping N/(m/s)  D_low=hs_damping N/(m/s)
      settings: InternalSimscapePortConfiguration="{\"Bottom\":[],\"Left\":[{\"id\":\"v\",\"label\":\"v\",\"type\":\"input\"},{\"id\":\"p\",\"label\":\"p\",\"type\":\"input\"}],\"Right\":[{\"id\":\"f\",\"label\":\"f\",\"type\":\"output\"}],\"Top\":[]}"
  PS Add Forces : fl_lib/Physical Signals/Functions/PS Add
  PS Gain Sign : fl_lib/Physical Signals/Functions/PS Gain  gain=-1
  v : PMIOPort  Side=Left
  p : PMIOPort  Port=2  Side=Left
  f : PMIOPort  Port=3  Side=Right
  connections:
  PS Gain Sign/LConn1 -- PS Add Forces/RConn1
  PS Add Forces/LConn1 -- Friction/RConn1
  PS Add Forces/LConn2 -- Hard Stop/RConn1
  Hard Stop/LConn1 -- v/RConn1 -- Friction/LConn1
  p/RConn1 -- Hard Stop/LConn2
  PS Gain Sign/RConn1 -- f/RConn1

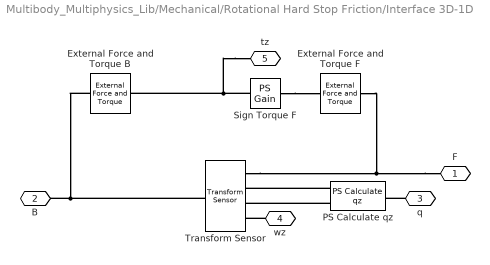
== system Multibody_Multiphysics_Lib/Mechanical/Rotational Hard Stop Friction/Interface 3D-1D ==
  External Force and Torque B : sm_lib/Forces and Torques/External Force and Torque  EnableForceX=off  EnableForceY=off  EnableForceZ=off  EnableForce=off  ForceResolutionFrame=AttachedFrame  EnableTorqueX=off  EnableTorqueY=off  EnableTorqueZ=on  EnableTorque=off  TorqueResolutionFrame=AttachedFrame
  External Force and Torque F : sm_lib/Forces and Torques/External Force and Torque  EnableForceX=off  EnableForceY=off  EnableForceZ=off  EnableForce=off  ForceResolutionFrame=AttachedFrame  EnableTorqueX=off  EnableTorqueY=off  EnableTorqueZ=on  EnableTorque=off  TorqueResolutionFrame=AttachedFrame
  PS Calculate qz : forcesPS_lib/Math/PS Calculate qz
      settings: InternalSimscapePortConfiguration="{\"Bottom\":[],\"Left\":[{\"id\":\"q\",\"label\":\"q\",\"type\":\"input\"},{\"id\":\"axs\",\"label\":\"axs\",\"type\":\"input\"}],\"Right\":[{\"id\":\"qz\",\"label\":\"qz\",\"type\":\"output\"}],\"Top\":[]}"
  Sign Torque F : fl_lib/Physical Signals/Functions/PS Gain  gain=-1
  Transform Sensor : sm_lib/Frames and Transforms/Transform Sensor  MeasurementFrame=Base  RotationSequence=XYX  SenseAngle=on  SenseAxis=on  SenseQ=off  SenseR=off  SenseRotationSequence=off  SenseOmegaX=off  SenseOmegaY=off  SenseOmegaZ=on  SenseOmega=off  SenseQDot=off  SenseRDot=off  SenseRotationSequenceDot=off  SenseAlphaX=off  SenseAlphaY=off  SenseAlphaZ=off  SenseAlpha=off  SenseQDDot=off  SenseRDDot=off  SenseX=off  SenseY=off  SenseZ=off  SenseXYZ=off  SenseRad=off  SenseAzim=off  SenseDist=off  SenseInc=off  SenseXDot=off  SenseYDot=off  SenseZDot=off  SenseXYZDot=off  SenseRadDot=off  SenseAzimDot=off  SenseDistDot=off  SenseIncDot=off  SenseXDDot=off  SenseYDDot=off  SenseZDDot=off  SenseXYZDDot=off  SenseRadDDot=off  SenseAzimDDot=off  SenseDistDDot=off  SenseIncDDot=off
  F : PMIOPort  Side=Right
  B : PMIOPort  Port=2  Side=Left
  q : PMIOPort  Port=3  Side=Left
  wz : PMIOPort  Port=4  Side=Left
  tz : PMIOPort  Port=5  Side=Right
  connections:
  q/RConn1 -- PS Calculate qz/RConn1
  PS Calculate qz/LConn2 -- Transform Sensor/RConn3
  PS Calculate qz/LConn1 -- Transform Sensor/RConn2
  tz/RConn1 -- External Force and Torque B/LConn1 -- Sign Torque F/LConn1
  Sign Torque F/RConn1 -- External Force and Torque F/LConn1
  wz/RConn1 -- Transform Sensor/RConn4
  External Force and Torque B/RConn1 -- B/RConn1 -- Transform Sensor/LConn1
  F/RConn1 -- Transform Sensor/RConn1 -- External Force and Torque F/RConn1

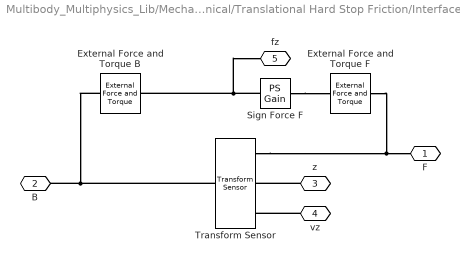
== system Multibody_Multiphysics_Lib/Mechanical/Translational Hard Stop Friction/Interface 3D-1D ==
  External Force and Torque B : sm_lib/Forces and Torques/External Force and Torque  EnableForceX=off  EnableForceY=off  EnableForceZ=on  EnableForce=off  ForceResolutionFrame=AttachedFrame  EnableTorqueX=off  EnableTorqueY=off  EnableTorqueZ=off  EnableTorque=off  TorqueResolutionFrame=AttachedFrame
  External Force and Torque F : sm_lib/Forces and Torques/External Force and Torque  EnableForceX=off  EnableForceY=off  EnableForceZ=on  EnableForce=off  ForceResolutionFrame=AttachedFrame  EnableTorqueX=off  EnableTorqueY=off  EnableTorqueZ=off  EnableTorque=off  TorqueResolutionFrame=AttachedFrame
  Sign Force F : fl_lib/Physical Signals/Functions/PS Gain  gain=-1
  Transform Sensor : sm_lib/Frames and Transforms/Transform Sensor  MeasurementFrame=Base  RotationSequence=XYX  SenseAngle=off  SenseAxis=off  SenseQ=off  SenseR=off  SenseRotationSequence=off  SenseOmegaX=off  SenseOmegaY=off  SenseOmegaZ=off  SenseOmega=off  SenseQDot=off  SenseRDot=off  SenseRotationSequenceDot=off  SenseAlphaX=off  SenseAlphaY=off  SenseAlphaZ=off  SenseAlpha=off  SenseQDDot=off  SenseRDDot=off  SenseX=off  SenseY=off  SenseZ=on  SenseXYZ=off  SenseRad=off  SenseAzim=off  SenseDist=off  SenseInc=off  SenseXDot=off  SenseYDot=off  SenseZDot=on  SenseXYZDot=off  SenseRadDot=off  SenseAzimDot=off  SenseDistDot=off  SenseIncDot=off  SenseXDDot=off  SenseYDDot=off  SenseZDDot=off  SenseXYZDDot=off  SenseRadDDot=off  SenseAzimDDot=off  SenseDistDDot=off  SenseIncDDot=off
  F : PMIOPort  Side=Right
  B : PMIOPort  Port=2  Side=Left
  z : PMIOPort  Port=3  Side=Left
  vz : PMIOPort  Port=4  Side=Left
  fz : PMIOPort  Port=5  Side=Right
  connections:
  Transform Sensor/RConn1 -- F/RConn1 -- External Force and Torque F/RConn1
  Transform Sensor/LConn1 -- B/RConn1 -- External Force and Torque B/RConn1
  z/RConn1 -- Transform Sensor/RConn2
  vz/RConn1 -- Transform Sensor/RConn3
  Sign Force F/RConn1 -- External Force and Torque F/LConn1
  Sign Force F/LConn1 -- External Force and Torque B/LConn1 -- fz/RConn1
